simulink model "Simulink_Master_AQUAHOLICS_ASV"  (R2026b)
settings: Solver=VariableStepAuto
settings Model: Creator=Dhaneshwara  LastModifiedBy=Dhaneshwara

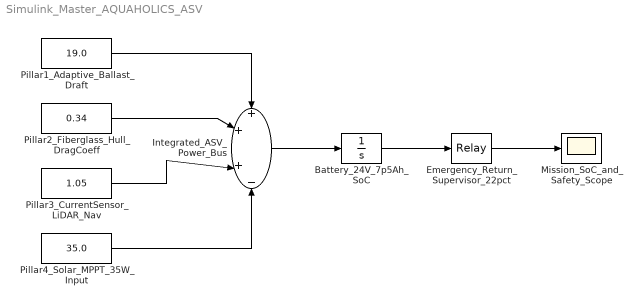
== system Simulink_Master_AQUAHOLICS_ASV ==
  Battery_24V_7p5Ah_SoC : Integrator  InitialCondition=100
  Emergency_Return_Supervisor_22pct : Relay  OnSwitchValue=35  OffSwitchValue=22
  Integrated_ASV_Power_Bus : Sum  Inputs=+++-
  Mission_SoC_and_Safety_Scope : Scope
  Pillar1_Adaptive_Ballast_Draft : Constant  Value=19.0
  Pillar2_Fiberglass_Hull_DragCoeff : Constant  Value=0.34
  Pillar3_CurrentSensor_LiDAR_Nav : Constant  Value=1.05
  Pillar4_Solar_MPPT_35W_Input : Constant  Value=35.0
  wires:
  Pillar1_Adaptive_Ballast_Draft/1 -> Integrated_ASV_Power_Bus/1
  Pillar2_Fiberglass_Hull_DragCoeff/1 -> Integrated_ASV_Power_Bus/2
  Pillar3_CurrentSensor_LiDAR_Nav/1 -> Integrated_ASV_Power_Bus/3
  Pillar4_Solar_MPPT_35W_Input/1 -> Integrated_ASV_Power_Bus/4
  Integrated_ASV_Power_Bus/1 -> Battery_24V_7p5Ah_SoC/1
  Battery_24V_7p5Ah_SoC/1 -> Emergency_Return_Supervisor_22pct/1
  Emergency_Return_Supervisor_22pct/1 -> Mission_SoC_and_Safety_Scope/1
